simulink model "suspensao_semiativa"  (R2024b)
settings: Solver=ode4  StartTime=0.0  StopTime=t_final  FixedStep=dt  RelTol=1e-3
PostLoadFcn:
  | addpath(fileparts(get_param(bdroot,'FileName'))); if evalin('base','exist(''Ts'',''var'')')==0, carregar_versao('v1'); end
values from neighbouring files (symbols this model uses):
  R = table(Ts_ms, tau_val_ms, sementes, a_pass, a_semi,      100*(a_semi./a_pass-1), carga_pass, carga_semi, 100*(carga_semi./carga_pass-1),      splitapply(@min, B.N_min_passivo_N, grupo), splitapply(@min, B.N_min_semi_N, grupo),      splitapply(@sum, ~B.contato_valido_passivo, grupo), splitapply(@sum, ~B.contato_valido_semi, grupo),      splitapply(@mean, B.tempo_N_nao_positivo_semi_s, grupo), splita ...(+372 chars)    [executar_v3_simulink.m]
undefined symbols (not defined in the file or in its folder): A_p, A_sd, B_p, B_sd, bias_ext, c_inicial, c_max, c_min, C_p, c_pass, C_sd, c_sky, D_p, D_sd, i0, i_max, K_a, K_ci, K_ext, K_v, K_vrel, Ki, Kp, L, tau_v, Ts, usar_sensores, v_eps, V_max, V_min
libraries: slpidlib x1
settings Model: Creator=muril  LastModifiedBy=muril

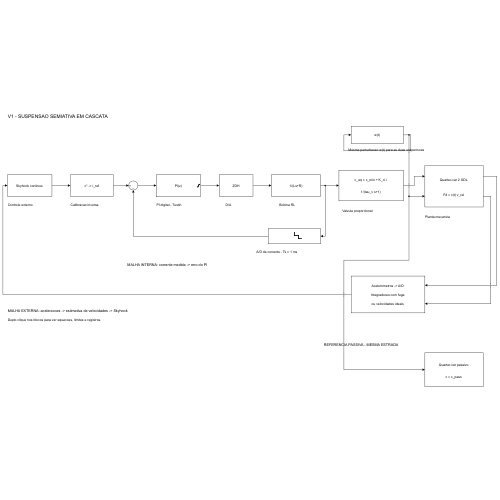
[thumbnail: Simulink's stored preview of the top-level diagram]
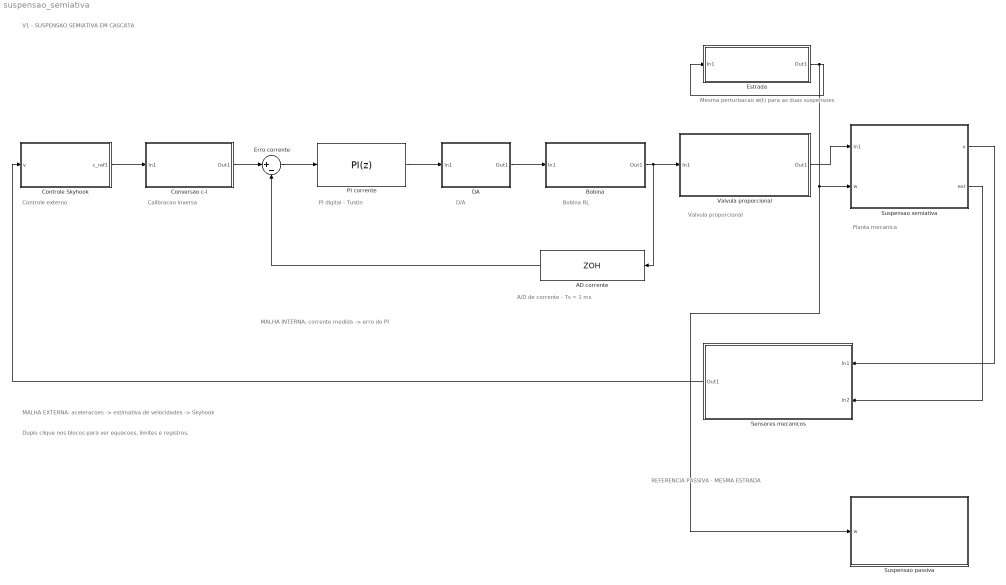
== system suspensao_semiativa ==
  note: V1 - SUSPENSAO SEMIATIVA EM CASCATA
  note: Mesma perturbacao w(t) para as duas suspensoes
  note: Controle externo
  note: Calibracao inversa
  note: PI digital - Tustin
  note: D/A
  note: Bobina RL
  note: Valvula proporcional
  note: Planta mecanica
  note: A/D de corrente - Ts = 1 ms
  note: MALHA INTERNA: corrente medida -> erro do PI
  note: MALHA EXTERNA: aceleracoes -> estimativa de velocidades -> Skyhook
  note: REFERENCIA PASSIVA - MESMA ESTRADA
  note: Duplo clique nos blocos para ver equacoes, limites e registros.
  AD corrente : ZeroOrderHold  SampleTime=Ts
  Bobina : Subsystem
      mask Display: disp('1/(Ls+R)');
  Controle Skyhook : Subsystem
      mask Display: disp('Skyhook continuo');
  Conversao c-i : Subsystem
      mask Display: disp('c* -> i_ref');
  DA : Subsystem
      mask Display: disp('ZOH');
  Erro corrente : Sum  Inputs=|+-
  Estrada : Subsystem
      mask Display: disp('w(t)');
  PI corrente : slpidlib/PID Controller  Controller=PI  Form=Parallel  TimeDomain=Discrete-time  UseExternalTs=off  SampleTime=Ts  IntegratorMethod=Trapezoidal  FilterMethod=Forward Euler  ControllerParametersSource=internal  P=Kp  I=Ki  UseKiTs=off  D=0  UseExternalDerivativeSource=off  N=100  UseFilter=on  TunerSelectOption=Transfer Function Based (PID Tuner App)  InitialConditionSource=internal  InitialConditionForIntegrator=R*i0  InitialConditionForFilter=0  DifferentiatorICPrevScaledInput=0  ExternalReset=none  TrackingMode=off  Kt=1  LimitOutput=on  SatLimitsSource=internal  UpperSaturationLimit=V_max  LowerSaturationLimit=V_min  LinearizeAsGain=off  AntiWindupMode=clamping  Kb=1  LimitIntegrator=off  UpperIntegratorSaturationLimit=inf  LowerIntegratorSaturationLimit=-inf  POutMin=[]  POutMax=[]  IOutMin=[]  IOutMax=[]  DOutMin=[]  DOutMax=[]  NOutMin=[]  NOutMax=[]  SumOutMin=[]  SumOutMax=[]  SaturationOutMin=[]  SaturationOutMax=[]  PParamMin=[]  PParamMax=[]  IParamMin=[]  IParamMax=[]  DParamMin=[]  DParamMax=[]  NParamMin=[]  NParamMax=[]  KbParamMin=[]  KbParamMax=[]  KtParamMin=[]  KtParamMax=[]  KbOutMin=[]  KbOutMax=[]  KtOutMin=[]  KtOutMax=[]  IntegratorOutMin=[]  IntegratorOutMax=[]  FilterOutMin=[]  FilterOutMax=[]  SumI1OutMin=[]  SumI1OutMax=[]  SumI2OutMin=[]  SumI2OutMax=[]  SumI3OutMin=[]  SumI3OutMax=[]  SumI4OutMin=[]  SumI4OutMax=[]  SumDOutMin=[]  SumDOutMax=[]  DifferentiatorOutMin=[]  DifferentiatorOutMax=[]  FilterDiffOutCoefMin=[]  FilterDiffOutCoefMax=[]  ReciprocalOutMin=[]  ReciprocalOutMax=[]  SumDenOutMin=[]  SumDenOutMax=[]  SumNumOutMin=[]  SumNumOutMax=[]  DivideOutMin=[]  DivideOutMax=[]  UdiffTsProdOutMin=[]  UdiffTsProdOutMax=[]  NTsProdOutMin=[]  NTsProdOutMax=[]  UintegralTsProdOutMin=[]  UintegralTsProdOutMax=[]  UngainTsProdOutMin=[]  UngainTsProdOutMax=[]  ClampingZeroOutDataTypeStr=Inherit: Inherit via back propagation  ClampingZeroOutMin=[]  ClampingZeroOutMax=[]  FilterDenConstantOutDataTypeStr=Inherit: Inherit via back propagation  FilterDenConstantOutMin=[]  FilterDenConstantOutMax=[]  PCopyOutDataTypeStr=Inherit: Inherit via back propagation  PCopyOutMin=[]  PCopyOutMax=[]  NCopyOutDataTypeStr=Inherit: Inherit via back propagation  NCopyOutMin=[]  NCopyOutMax=[]  IntegratorContinuousStateAttributes=''  IntegratorStateMustResolveToSignalObject=off  IntegratorRTWStateStorageClass=Auto  FilterContinuousStateAttributes=''  FilterStateMustResolveToSignalObject=off  FilterRTWStateStorageClass=Auto  ParallelPVariant=InternalParameters  IdealPVariant=Disabled  IVariant=InternalParameters  DVariant=Disabled  IntegratorVariant=Discrete  SatVariant=Enabled  AWVariant=DiscClampingParallel  PCopyVariant=Disabled  TRVariant=Disabled  FdbkBlocksVariant=Feedback  IdealPFdbkVariant=Passthrough  SatFdbkVariant=Passthrough  DerivativeFilterVariant=Disabled  NVariant=Disabled  NCopyVariant=Disabled_SignalSpec  FilterICVariant=Disabled  IntegratorICVariant=InternalICs  ExternalResetVariant=Disabled  TRSumVariant=Passthrough  SumFdbkVariant=Enabled  SumVariant=Sum_PI  TsampFilterVariant=InternalTs  TsampNgainVariant=Passthrough  TsampIntegralVariant=Disabled_SignalSpec  ExternalSaturationOutDataTypeStr=Inherit: Same as second input  DerivativeSourceVariant=Disabled  PreIntVariant=InternalPreInt
      settings: LibrarySourceBlock=simulink/Discrete/Discrete PID Controller
  Sensores mecanicos : Subsystem
      mask Display: text(0.5,0.75,'Acelerometros -> A/D','horizontalAlignment','center'); text(0.5,0.5,'Integradores com fuga','horizontalAlignment','center'); text(0.5,0.25,'ou velocidades ideais','horizontalAlignment','center');
  Suspensao passiva : Subsystem
      mask Display: text(0.5,0.65,'Quarter-car passivo','horizontalAlignment','center'); text(0.5,0.3,'c = c_pass','horizontalAlignment','center');
  Suspensao semiativa : Subsystem
      mask Display: text(0.5,0.65,'Quarter-car 2 GDL','horizontalAlignment','center'); text(0.5,0.3,'Fd = c(t) v_rel','horizontalAlignment','center');
  Valvula proporcional : Subsystem
      mask Display: text(0.5,0.7,'c_eq = c_min + K_ci i','horizontalAlignment','center'); text(0.5,0.3,'1/(tau_v s+1)','horizontalAlignment','center');
  wires:
  AD corrente/1 -> Erro corrente/2
  Erro corrente/1 -> PI corrente/1
  Estrada/1(Out1) -> Suspensao semiativa/2(w), Suspensao passiva/1(w), Estrada/1(In1)
  Suspensao semiativa/1(x) -> Sensores mecanicos/1(In1)
  Suspensao semiativa/2(ext) -> Sensores mecanicos/2(In2)
  Sensores mecanicos/1(Out1) -> Controle Skyhook/1(v)
  Controle Skyhook/1(c_ref1) -> Conversao c-i/1(In1)
  Conversao c-i/1(Out1) -> Erro corrente/1
  Valvula proporcional/1(Out1) -> Suspensao semiativa/1(In1)
  Bobina/1(Out1) -> Valvula proporcional/1(In1), AD corrente/1
  PI corrente/1 -> DA/1(In1)
  DA/1(Out1) -> Bobina/1(In1)

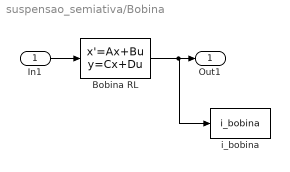
== system suspensao_semiativa/Bobina ==
  In1 : Inport
  Bobina RL : StateSpace  A=-R/L  B=1/L  D=0  InitialCondition=i0
  i_bobina : ToWorkspace  VariableName=i_bobina  SaveFormat=Timeseries  SampleTime=-1
  Out1 : Outport
  wires:
  Bobina RL/1 -> i_bobina/1, Out1/1
  In1/1 -> Bobina RL/1

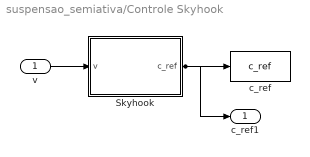
== system suspensao_semiativa/Controle Skyhook ==
  v : Inport
  Skyhook : MATLAB Function  TreatAsAtomicUnit=on
  c_ref : ToWorkspace  VariableName=c_ref  SaveFormat=Timeseries  SampleTime=-1
  c_ref1 : Outport
  wires:
  Skyhook/1(c_ref) -> c_ref1/1, c_ref/1
  v/1 -> Skyhook/1(v)

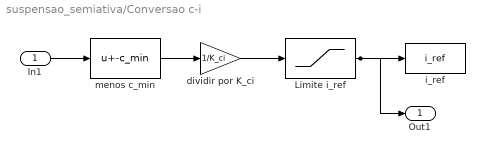
== system suspensao_semiativa/Conversao c-i ==
  In1 : Inport
  Limite i_ref : Saturate  UpperLimit=i_max  LowerLimit=0
  dividir por K_ci : Gain  Gain=1/K_ci
  i_ref : ToWorkspace  VariableName=i_ref  SaveFormat=Timeseries  SampleTime=-1
  menos c_min : Bias  Bias=-c_min  SaturateOnIntegerOverflow=off
  Out1 : Outport
  wires:
  In1/1 -> menos c_min/1
  menos c_min/1 -> dividir por K_ci/1
  dividir por K_ci/1 -> Limite i_ref/1
  Limite i_ref/1 -> i_ref/1, Out1/1

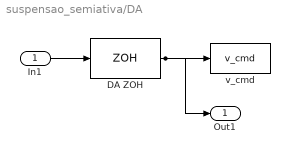
== system suspensao_semiativa/DA ==
  In1 : Inport
  DA ZOH : ZeroOrderHold  SampleTime=Ts
  v_cmd : ToWorkspace  VariableName=v_cmd  SaveFormat=Timeseries  SampleTime=-1
  Out1 : Outport
  wires:
  In1/1 -> DA ZOH/1
  DA ZOH/1 -> v_cmd/1, Out1/1

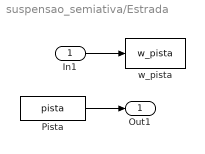
== system suspensao_semiativa/Estrada ==
  In1 : Inport
  Pista : FromWorkspace  VariableName=pista  OutputAfterFinalValue=Holding final value
  w_pista : ToWorkspace  VariableName=w_pista  SaveFormat=Timeseries  SampleTime=-1
  Out1 : Outport
  wires:
  In1/1 -> w_pista/1
  Pista/1 -> Out1/1

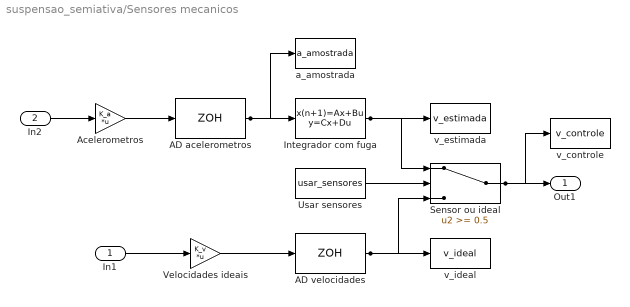
== system suspensao_semiativa/Sensores mecanicos ==
  In1 : Inport
  In2 : Inport  Port=2
  AD acelerometros : ZeroOrderHold  SampleTime=Ts
  AD velocidades : ZeroOrderHold  SampleTime=Ts
  Acelerometros : Gain  Gain=K_a  Multiplication=Matrix(K*u)
  Integrador com fuga : DiscreteStateSpace  A=A_sd  B=B_sd  C=C_sd  D=D_sd  InitialCondition=zeros(2,1)  SampleTime=Ts
  Sensor ou ideal : Switch  Threshold=0.5  SaturateOnIntegerOverflow=off  InputSameDT=off
  Usar sensores : Constant  Value=usar_sensores
  Velocidades ideais : Gain  Gain=K_v  Multiplication=Matrix(K*u)
  a_amostrada : ToWorkspace  VariableName=a_amostrada  SaveFormat=Timeseries  SampleTime=-1
  v_controle : ToWorkspace  VariableName=v_controle  SaveFormat=Timeseries  SampleTime=-1
  v_estimada : ToWorkspace  VariableName=v_estimada  SaveFormat=Timeseries  SampleTime=-1
  v_ideal : ToWorkspace  VariableName=v_ideal  SaveFormat=Timeseries  SampleTime=-1
  Out1 : Outport
  wires:
  In2/1 -> Acelerometros/1
  Velocidades ideais/1 -> AD velocidades/1
  Acelerometros/1 -> AD acelerometros/1
  In1/1 -> Velocidades ideais/1
  AD velocidades/1 -> v_ideal/1, Sensor ou ideal/3
  AD acelerometros/1 -> a_amostrada/1, Integrador com fuga/1
  Integrador com fuga/1 -> v_estimada/1, Sensor ou ideal/1
  Usar sensores/1 -> Sensor ou ideal/2
  Sensor ou ideal/1 -> v_controle/1, Out1/1

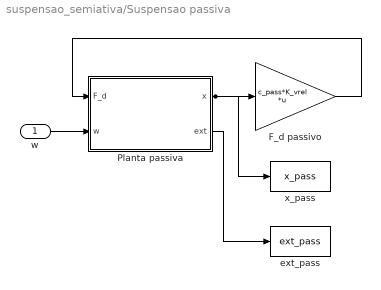
== system suspensao_semiativa/Suspensao passiva ==
  w : Inport
  F_d passivo : Gain  Gain=c_pass*K_vrel  Multiplication=Matrix(K*u)
  Planta passiva : Subsystem
  ext_pass : ToWorkspace  VariableName=ext_pass  SaveFormat=Timeseries  SampleTime=-1
  x_pass : ToWorkspace  VariableName=x_pass  SaveFormat=Timeseries  SampleTime=-1
  wires:
  w/1 -> Planta passiva/2(w)
  Planta passiva/1(x) -> F_d passivo/1, x_pass/1
  F_d passivo/1 -> Planta passiva/1(F_d)
  Planta passiva/2(ext) -> ext_pass/1

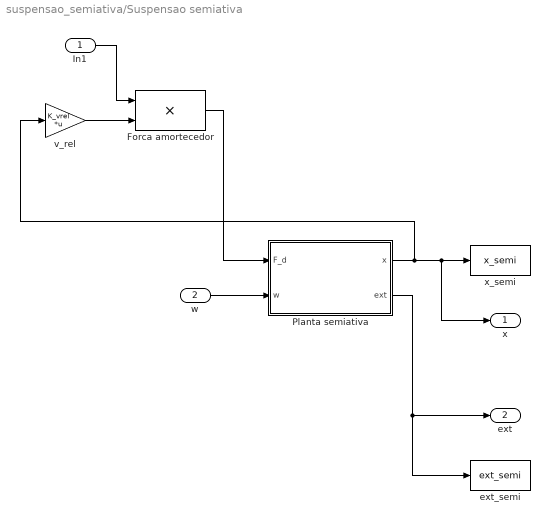
== system suspensao_semiativa/Suspensao semiativa ==
  In1 : Inport
  w : Inport  Port=2
  Forca amortecedor : Product
  Planta semiativa : Subsystem
  ext_semi : ToWorkspace  VariableName=ext_semi  SaveFormat=Timeseries  SampleTime=-1
  v_rel : Gain  Gain=K_vrel  Multiplication=Matrix(K*u)
  x_semi : ToWorkspace  VariableName=x_semi  SaveFormat=Timeseries  SampleTime=-1
  x : Outport
  ext : Outport  Port=2
  wires:
  Forca amortecedor/1 -> Planta semiativa/1(F_d)
  v_rel/1 -> Forca amortecedor/2
  w/1 -> Planta semiativa/2(w)
  Planta semiativa/2(ext) -> ext/1, ext_semi/1
  Planta semiativa/1(x) -> x/1, x_semi/1, v_rel/1
  In1/1 -> Forca amortecedor/1

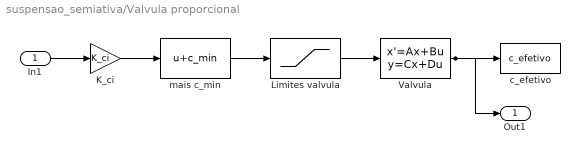
== system suspensao_semiativa/Valvula proporcional ==
  In1 : Inport
  K_ci : Gain  Gain=K_ci
  Limites valvula : Saturate  UpperLimit=c_max  LowerLimit=c_min
  Valvula : StateSpace  A=-1/tau_v  B=1/tau_v  D=0  InitialCondition=c_inicial
  c_efetivo : ToWorkspace  VariableName=c_efetivo  SaveFormat=Timeseries  SampleTime=-1
  mais c_min : Bias  Bias=c_min  SaturateOnIntegerOverflow=off
  Out1 : Outport
  wires:
  K_ci/1 -> mais c_min/1
  In1/1 -> K_ci/1
  mais c_min/1 -> Limites valvula/1
  Limites valvula/1 -> Valvula/1
  Valvula/1 -> c_efetivo/1, Out1/1

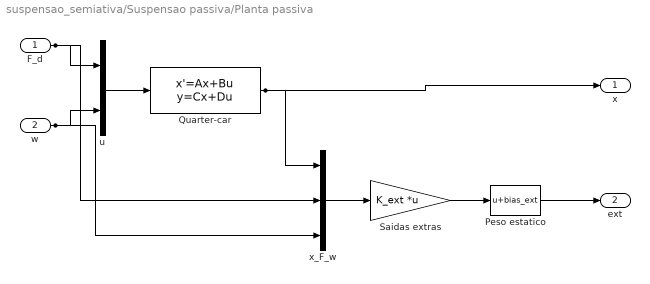
== system suspensao_semiativa/Suspensao passiva/Planta passiva ==
  F_d : Inport
  w : Inport  Port=2
  Peso estatico : Bias  Bias=bias_ext  SaturateOnIntegerOverflow=off
  Quarter-car : StateSpace  A=A_p  B=B_p  C=C_p  D=D_p  InitialCondition=zeros(4,1)
  Saidas extras : Gain  Gain=K_ext  Multiplication=Matrix(K*u)
  u : Mux  Inputs=2
  x_F_w : Mux  Inputs=3
  x : Outport
  ext : Outport  Port=2
  wires:
  F_d/1 -> u/1, x_F_w/2
  w/1 -> u/2, x_F_w/3
  u/1 -> Quarter-car/1
  Quarter-car/1 -> x/1, x_F_w/1
  x_F_w/1 -> Saidas extras/1
  Saidas extras/1 -> Peso estatico/1
  Peso estatico/1 -> ext/1

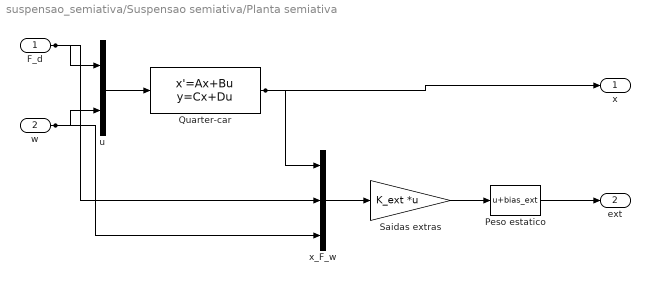
== system suspensao_semiativa/Suspensao semiativa/Planta semiativa ==
  F_d : Inport
  w : Inport  Port=2
  Peso estatico : Bias  Bias=bias_ext  SaturateOnIntegerOverflow=off
  Quarter-car : StateSpace  A=A_p  B=B_p  C=C_p  D=D_p  InitialCondition=zeros(4,1)
  Saidas extras : Gain  Gain=K_ext  Multiplication=Matrix(K*u)
  u : Mux  Inputs=2
  x_F_w : Mux  Inputs=3
  x : Outport
  ext : Outport  Port=2
  wires:
  F_d/1 -> u/1, x_F_w/2
  w/1 -> u/2, x_F_w/3
  u/1 -> Quarter-car/1
  Quarter-car/1 -> x/1, x_F_w/1
  x_F_w/1 -> Saidas extras/1
  Saidas extras/1 -> Peso estatico/1
  Peso estatico/1 -> ext/1

== matlab function suspensao_semiativa/Controle Skyhook/Skyhook ==
  data: v input; c_ref output; c_sky parameter; c_min parameter; c_max parameter; v_eps parameter
function c_ref = skyhook(v, c_sky, c_min, c_max, v_eps)
% v = [v_s; v_u] medidos. Saida: amortecimento pedido c*.
v_s = v(1);
v_rel = v(1) - v(2);
if v_s*v_rel <= 0
    % amortecedor atrapalharia: fica o mais macio possivel
    c_ref = c_min;
else
    c_ref = c_sky*v_s*v_rel/(v_rel^2 + v_eps^2);
    c_ref = min(max(c_ref, c_min), c_max);
end
